simulink model "AXU5EV_Encoder_Feedback"  (R2026b)
settings: Solver=FixedStepDiscrete  FixedStep=100e-6
libraries: AXU5EV_Encoder_Components x1
settings Model: Creator=lww  LastModifiedBy=lww
settings OptimizationCC: DefaultParameterBehavior=Inlined  DifferentSizesBufferReuse=on  EfficientTunableParamExpr=on  EnhancedBackFolding=on  OptimizationCustomize=off  OptimizeBlockOrder=speed  PassReuseOutputArgsAs=Individual arguments  RemoveInternalMemoryZeroInit=on  RemoveRootLevelIOMemoryZeroInit=on
settings DebuggingCC: ParameterTunabilityLossMsg=error
settings HardwareCC: ProdHWDeviceType=ARM Compatible->ARM Cortex-R  ProdLargestAtomicFloat=Double  ProdLargestAtomicInteger=Long  ProdLongLongMode=on
settings SFSimCC: MATLABDynamicMemAlloc=off
settings RTWCC: DataTypeReplacement=CDataTypesFixedWidth  Description=Embedded Coder  GenCodeOnly=on  SystemTargetFile=ert.tlc  TemplateMakefile=ert_default_tmf
settings CodeAppCC: ForceParamTrailComments=on  IgnoreCustomStorageClasses=off  InsertBlockDesc=on  OperatorAnnotations=on  SFDataObjDesc=on  SimulinkDataObjDesc=on
settings ERTTargetCC: CombineSignalStateStructs=on  GenerateSampleERTMain=on  MaxIdInt16=INT16_MAX  MaxIdInt32=INT32_MAX  MaxIdInt64=INT64_MAX  MaxIdInt8=INT8_MAX  MaxIdUint16=UINT16_MAX  MaxIdUint32=UINT32_MAX  MaxIdUint64=UINT64_MAX  MaxIdUint8=UINT8_MAX  MinIdInt16=INT16_MIN  MinIdInt32=INT32_MIN  MinIdInt64=INT64_MIN  MinIdInt8=INT8_MIN

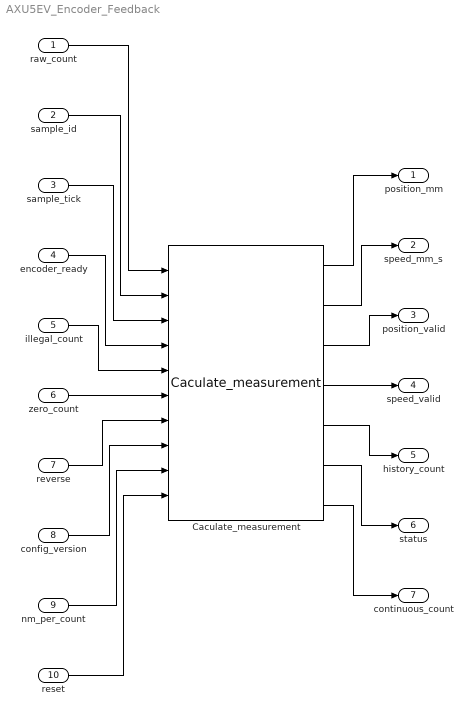
== system AXU5EV_Encoder_Feedback ==
  raw_count : Inport  OutDataTypeStr=uint32  SampleTime=100e-6  Interpolate=off
  sample_id : Inport  Port=2  OutDataTypeStr=uint32  SampleTime=100e-6  Interpolate=off
  sample_tick : Inport  Port=3  OutDataTypeStr=uint64  SampleTime=100e-6  Interpolate=off
  encoder_ready : Inport  Port=4  OutDataTypeStr=boolean  SampleTime=100e-6  Interpolate=off
  illegal_count : Inport  Port=5  OutDataTypeStr=uint32  SampleTime=100e-6  Interpolate=off
  zero_count : Inport  Port=6  OutDataTypeStr=uint32  SampleTime=100e-6  Interpolate=off
  reverse : Inport  Port=7  OutDataTypeStr=boolean  SampleTime=100e-6  Interpolate=off
  config_version : Inport  Port=8  OutDataTypeStr=uint32  SampleTime=100e-6  Interpolate=off
  nm_per_count : Inport  Port=9  OutDataTypeStr=uint32  SampleTime=100e-6  Interpolate=off
  reset : Inport  Port=10  OutDataTypeStr=boolean  SampleTime=100e-6  Interpolate=off
  Caculate_measurement : AXU5EV_Encoder_Components/Caculate_measurement  SystemSampleTime=-1  VariantActivationTime=update diagram  EmptyChoice=off  PassThrough=off  PassThroughVariantControl=(default)  EmptyChoiceVariantControl=(default)  AllowFlexibleInterface=on  Latency=0  AutoFrameSizeCalculation=off
  position_mm : Outport  OutDataTypeStr=double
  speed_mm_s : Outport  Port=2  OutDataTypeStr=double
  position_valid : Outport  Port=3  OutDataTypeStr=boolean
  speed_valid : Outport  Port=4  OutDataTypeStr=boolean
  history_count : Outport  Port=5  OutDataTypeStr=uint8
  status : Outport  Port=6  OutDataTypeStr=uint32
  continuous_count : Outport  Port=7  OutDataTypeStr=int64
  wires:
  Caculate_measurement/7 -> continuous_count/1
  Caculate_measurement/6 -> status/1
  Caculate_measurement/5 -> history_count/1
  Caculate_measurement/4 -> speed_valid/1
  Caculate_measurement/3 -> position_valid/1
  Caculate_measurement/2 -> speed_mm_s/1
  Caculate_measurement/1 -> position_mm/1
  reset/1 -> Caculate_measurement/10
  nm_per_count/1 -> Caculate_measurement/9
  config_version/1 -> Caculate_measurement/8
  reverse/1 -> Caculate_measurement/7
  zero_count/1 -> Caculate_measurement/6
  illegal_count/1 -> Caculate_measurement/5
  encoder_ready/1 -> Caculate_measurement/4
  sample_tick/1 -> Caculate_measurement/3
  sample_id/1 -> Caculate_measurement/2
  raw_count/1 -> Caculate_measurement/1
